simulink model "cravo_e_canela"  (R2024b)
settings: Solver=VariableStepAuto  StartTime=0.0  StopTime=simTim  RelTol=1e-3
libraries: commrfcorlib x2, audiodynamicrange x2, dspvision x1
settings Model: Creator=Pedro  LastModifiedBy=Pedro

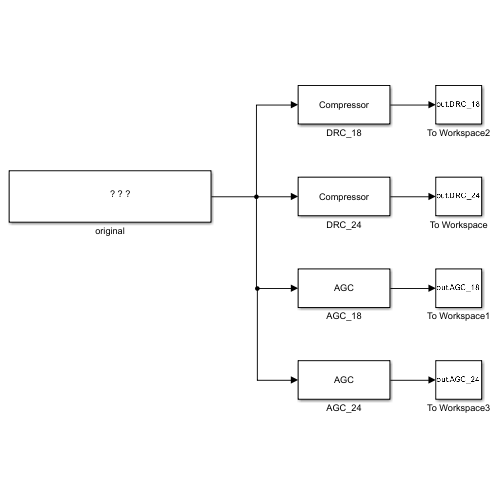
[thumbnail: Simulink's stored preview of the top-level diagram]
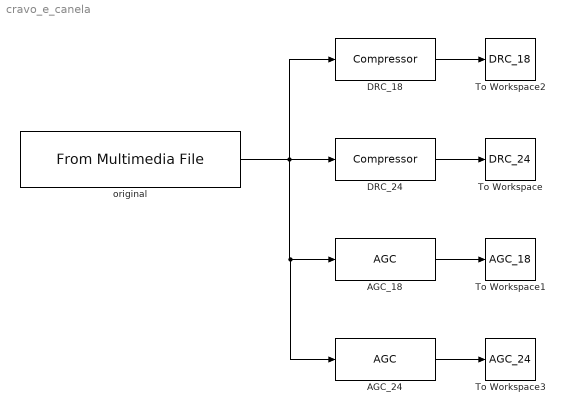
== system cravo_e_canela ==
  AGC_18 : commrfcorlib/AGC  LegacyMode=off  DetectorMethod=Rectifier  LoopMethod=Linear  UpdatePeriod=100  StepSize=0.1  AdaptationStepSize=AGC_Step_Size  DesiredOutputPower=10^(-18/10)  AveragingLength=AGC_Averging_Window_Length  MaximumGain=30  MaxPowerGain=AGC_Maximum_Power_Gain  GainOutputPort=off  InputPowerOutputPort=off  SimulateUsing=Code generation
  AGC_24 : commrfcorlib/AGC  LegacyMode=off  DetectorMethod=Rectifier  LoopMethod=Linear  UpdatePeriod=100  StepSize=0.1  AdaptationStepSize=AGC_Step_Size  DesiredOutputPower=10^(-24/10)  AveragingLength=AGC_Averging_Window_Length  MaximumGain=30  MaxPowerGain=AGC_Maximum_Power_Gain  GainOutputPort=off  InputPowerOutputPort=off  SimulateUsing=Code generation
  DRC_18 : audiodynamicrange/Compressor  ThresholdPort=off  Threshold=-18  RatioPort=off  Ratio=DRC_Ratio  KneeWidthPort=off  KneeWidth=DRC_Knee_Width  AttackTimePort=off  AttackTime=DRC_Attack_Time  ReleaseTimePort=off  ReleaseTime=DRC_Release_Time  MakeUpGainMode=Property  MakeUpGain=DRC_Make_up_Gain  InheritSampleRate=off  SampleRate=fs  outputGain=off  EnableSidechain=off  SimulateUsing=Interpreted execution
  DRC_24 : audiodynamicrange/Compressor  ThresholdPort=off  Threshold=-24  RatioPort=off  Ratio=DRC_Ratio  KneeWidthPort=off  KneeWidth=DRC_Knee_Width  AttackTimePort=off  AttackTime=DRC_Attack_Time  ReleaseTimePort=off  ReleaseTime=DRC_Release_Time  MakeUpGainMode=Property  MakeUpGain=DRC_Make_up_Gain  InheritSampleRate=off  SampleRate=fs  outputGain=off  EnableSidechain=off  SimulateUsing=Interpreted execution
  To Workspace : ToWorkspace  VariableName=DRC_24  SampleTime=-1
      settings: Save2DSignal=2-D array (concatenate along first dimension)
  To Workspace1 : ToWorkspace  VariableName=AGC_18  SampleTime=-1
      settings: Save2DSignal=2-D array (concatenate along first dimension)
  To Workspace2 : ToWorkspace  VariableName=DRC_18  SampleTime=-1
      settings: Save2DSignal=2-D array (concatenate along first dimension)
  To Workspace3 : ToWorkspace  VariableName=AGC_24  SampleTime=-1
      settings: Save2DSignal=2-D array (concatenate along first dimension)
  original : dspvision/From Multimedia File  inputFilename=input_path  readRange=[1 Inf]  loop=on  numPlays=1  outputStreams=Audio only  videoDataType=single  audioDataType=double  inheritSampleTime=on  userDefinedSampleTime=1/30  noAudioOutput=off  isIntensityVideo=off  fourcc=RGB  colorVideoFormat=Separate color signals  outputEOF=off  dataOrg=Column-major  audioFrameSize=1024  computeAudioFrameSize=off  outSamplingMode=Sample based
      settings: LibrarySourceBlock=audiosources/From Multimedia File
  wires:
  DRC_24/1 -> To Workspace/1
  AGC_18/1 -> To Workspace1/1
  original/1 -> DRC_18/1, AGC_24/1, AGC_18/1, DRC_24/1
  DRC_18/1 -> To Workspace2/1
  AGC_24/1 -> To Workspace3/1
